simulink model "r23_512p_fft"  (R2026b)
settings: Solver=FixedStepDiscrete  StopTime=5e-5*(127-1)  FixedStep=5e-5
libraries: dspsrcs4 x8
(part 1 of 3)
settings Model: Creator=bzwang_admin  LastModifiedBy=bzwang
settings OptimizationCC: BlockReduction=off  ConditionallyExecuteInputs=off  DefaultParameterBehavior=Inlined  OptimizeBlockIOStorage=off
settings HardwareCC: ProdEndianess=Unspecified  ProdEqTarget=off  ProdHWDeviceType=ASIC/FPGA->ASIC/FPGA  ProdIntDivRoundTo=Undefined  ProdLargestAtomicFloat=None  TargetEndianess=LittleEndian  TargetHWDeviceType=Custom Processor->MATLAB Host Computer  TargetIntDivRoundTo=Zero  TargetLongLongMode=on
settings RTWCC: GenerateReport=on  LaunchReport=on  PackageGeneratedCodeAndArtifacts=on
settings CodeAppCC: ForceParamTrailComments=on  MATLABSourceComments=on  StateflowObjectComments=on

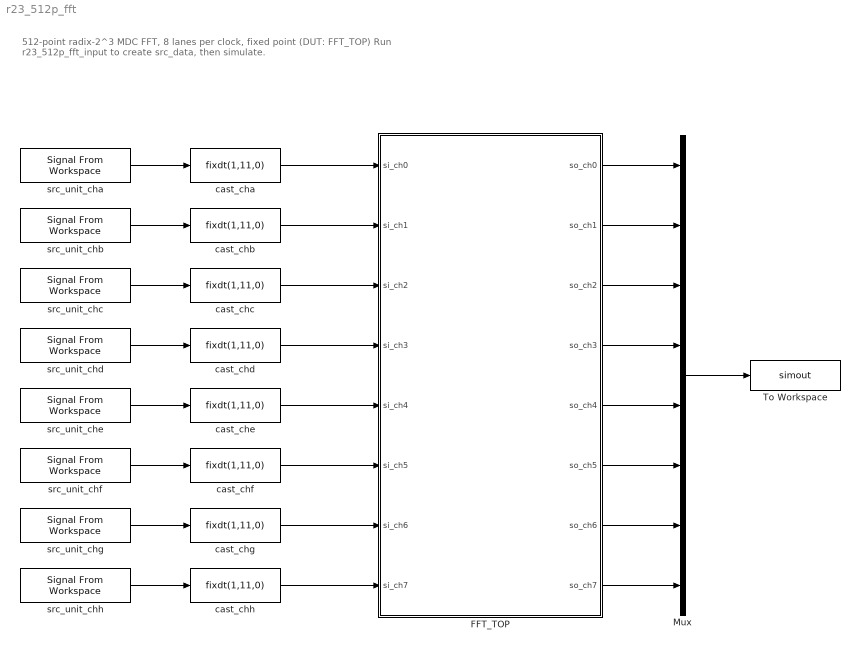
== system r23_512p_fft ==
  note: 512-point radix-2^3 MDC FFT, 8 lanes per clock, fixed point (DUT: FFT_TOP)
      | Run r23_512p_fft_input to create src_data, then simulate.
  FFT_TOP : Subsystem  TreatAsAtomicUnit=on
  Mux : Mux  Inputs=8
  To Workspace : ToWorkspace  VariableName=simout  SampleTime=-1
  cast_cha : DataTypeConversion  OutDataTypeStr=fixdt(1,11,0)  SaturateOnIntegerOverflow=off  RndMeth=Floor
  cast_chb : DataTypeConversion  OutDataTypeStr=fixdt(1,11,0)  SaturateOnIntegerOverflow=off  RndMeth=Floor
  cast_chc : DataTypeConversion  OutDataTypeStr=fixdt(1,11,0)  SaturateOnIntegerOverflow=off  RndMeth=Floor
  cast_chd : DataTypeConversion  OutDataTypeStr=fixdt(1,11,0)  SaturateOnIntegerOverflow=off  RndMeth=Floor
  cast_che : DataTypeConversion  OutDataTypeStr=fixdt(1,11,0)  SaturateOnIntegerOverflow=off  RndMeth=Floor
  cast_chf : DataTypeConversion  OutDataTypeStr=fixdt(1,11,0)  SaturateOnIntegerOverflow=off  RndMeth=Floor
  cast_chg : DataTypeConversion  OutDataTypeStr=fixdt(1,11,0)  SaturateOnIntegerOverflow=off  RndMeth=Floor
  cast_chh : DataTypeConversion  OutDataTypeStr=fixdt(1,11,0)  SaturateOnIntegerOverflow=off  RndMeth=Floor
  src_unit_cha : dspsrcs4/Signal From Workspace  X=src_data.cha  Ts=5e-5  nsamps=1  OutputAfterFinalValue=Setting to zero  ignoreOrWarnInputAndFrameLengths=off  OutputFrames=off
  src_unit_chb : dspsrcs4/Signal From Workspace  X=src_data.chb  Ts=5e-5  nsamps=1  OutputAfterFinalValue=Setting to zero  ignoreOrWarnInputAndFrameLengths=off  OutputFrames=off
  src_unit_chc : dspsrcs4/Signal From Workspace  X=src_data.chc  Ts=5e-5  nsamps=1  OutputAfterFinalValue=Setting to zero  ignoreOrWarnInputAndFrameLengths=off  OutputFrames=off
  src_unit_chd : dspsrcs4/Signal From Workspace  X=src_data.chd  Ts=5e-5  nsamps=1  OutputAfterFinalValue=Setting to zero  ignoreOrWarnInputAndFrameLengths=off  OutputFrames=off
  src_unit_che : dspsrcs4/Signal From Workspace  X=src_data.che  Ts=5e-5  nsamps=1  OutputAfterFinalValue=Setting to zero  ignoreOrWarnInputAndFrameLengths=off  OutputFrames=off
  src_unit_chf : dspsrcs4/Signal From Workspace  X=src_data.chf  Ts=5e-5  nsamps=1  OutputAfterFinalValue=Setting to zero  ignoreOrWarnInputAndFrameLengths=off  OutputFrames=off
  src_unit_chg : dspsrcs4/Signal From Workspace  X=src_data.chg  Ts=5e-5  nsamps=1  OutputAfterFinalValue=Setting to zero  ignoreOrWarnInputAndFrameLengths=off  OutputFrames=off
  src_unit_chh : dspsrcs4/Signal From Workspace  X=src_data.chh  Ts=5e-5  nsamps=1  OutputAfterFinalValue=Setting to zero  ignoreOrWarnInputAndFrameLengths=off  OutputFrames=off
  wires:
  src_unit_cha/1 -> cast_cha/1
  cast_cha/1 -> FFT_TOP/1(si_ch0)
  FFT_TOP/1(so_ch0) -> Mux/1
  src_unit_chb/1 -> cast_chb/1
  cast_chb/1 -> FFT_TOP/2(si_ch1)
  FFT_TOP/2(so_ch1) -> Mux/2
  src_unit_chc/1 -> cast_chc/1
  cast_chc/1 -> FFT_TOP/3(si_ch2)
  FFT_TOP/3(so_ch2) -> Mux/3
  src_unit_chd/1 -> cast_chd/1
  cast_chd/1 -> FFT_TOP/4(si_ch3)
  FFT_TOP/4(so_ch3) -> Mux/4
  src_unit_che/1 -> cast_che/1
  cast_che/1 -> FFT_TOP/5(si_ch4)
  FFT_TOP/5(so_ch4) -> Mux/5
  src_unit_chf/1 -> cast_chf/1
  cast_chf/1 -> FFT_TOP/6(si_ch5)
  FFT_TOP/6(so_ch5) -> Mux/6
  src_unit_chg/1 -> cast_chg/1
  cast_chg/1 -> FFT_TOP/7(si_ch6)
  FFT_TOP/7(so_ch6) -> Mux/7
  src_unit_chh/1 -> cast_chh/1
  cast_chh/1 -> FFT_TOP/8(si_ch7)
  FFT_TOP/8(so_ch7) -> Mux/8
  Mux/1 -> To Workspace/1

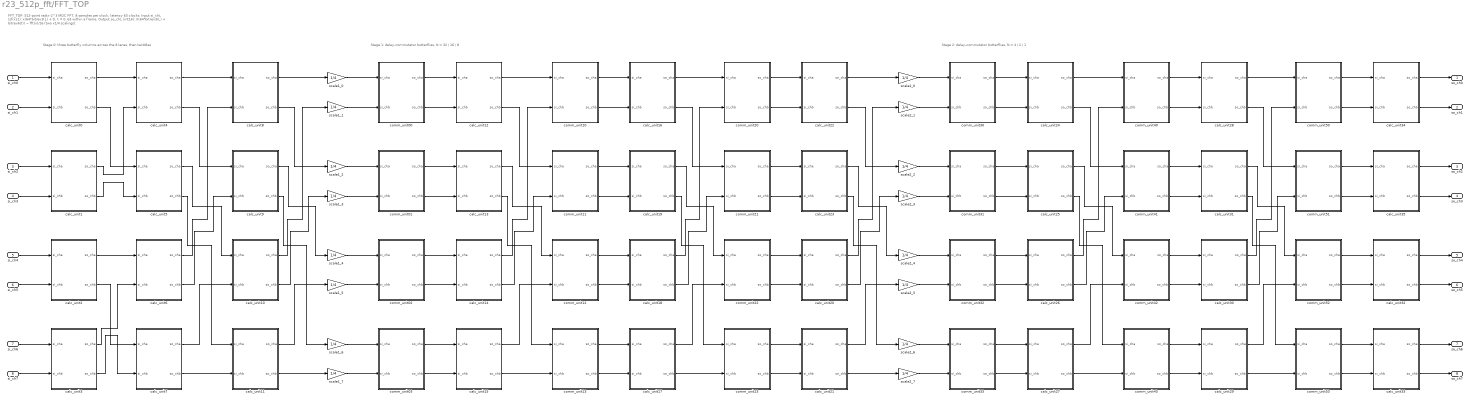
== system r23_512p_fft/FFT_TOP ==
  note: Stage 2: delay-commutator butterflies, N = 4 / 2 / 1
  note: Stage 1: delay-commutator butterflies, N = 32 / 16 / 8
  note: Stage 0: three butterfly columns across the 8 lanes, then twiddles
  note: FFT_TOP: 512-point radix-2^3 MDC FFT, 8 samples per clock, latency 63 clocks.
      | Input  si_chL (sfix11): x(64*bitrev3(L) + t), t = 0..63 within a frame.
      | Output so_chL (int16):  X(64*bitrev3(L) + bitrev6(t)) ~ fft(x)/16 (two x1/4 scalings).
  si_ch0 : Inport
  si_ch1 : Inport  Port=2
  si_ch2 : Inport  Port=3
  si_ch3 : Inport  Port=4
  si_ch4 : Inport  Port=5
  si_ch5 : Inport  Port=6
  si_ch6 : Inport  Port=7
  si_ch7 : Inport  Port=8
  calc_unit0 : Subsystem
  calc_unit1 : Subsystem
  calc_unit10 : Subsystem
  calc_unit11 : Subsystem
  calc_unit12 : Subsystem
  calc_unit13 : Subsystem
  calc_unit14 : Subsystem
  calc_unit15 : Subsystem
  calc_unit16 : Subsystem
  calc_unit17 : Subsystem
  calc_unit18 : Subsystem
  calc_unit19 : Subsystem
  calc_unit2 : Subsystem
  calc_unit20 : Subsystem
  calc_unit21 : Subsystem
  calc_unit22 : Subsystem
  calc_unit23 : Subsystem
  calc_unit24 : Subsystem
  calc_unit25 : Subsystem
  calc_unit26 : Subsystem
  calc_unit27 : Subsystem
  calc_unit28 : Subsystem
  calc_unit29 : Subsystem
  calc_unit3 : Subsystem
  calc_unit30 : Subsystem
  calc_unit31 : Subsystem
  calc_unit32 : Subsystem
  calc_unit33 : Subsystem
  calc_unit34 : Subsystem
  calc_unit35 : Subsystem
  calc_unit4 : Subsystem
  calc_unit5 : Subsystem
  calc_unit6 : Subsystem
  calc_unit7 : Subsystem
  calc_unit8 : Subsystem
  calc_unit9 : Subsystem
  comm_unit00 : Subsystem
      settings: AttributesFormatString=N = 32
  comm_unit01 : Subsystem
      settings: AttributesFormatString=N = 32
  comm_unit02 : Subsystem
      settings: AttributesFormatString=N = 32
  comm_unit03 : Subsystem
      settings: AttributesFormatString=N = 32
  comm_unit10 : Subsystem
      settings: AttributesFormatString=N = 16
  comm_unit11 : Subsystem
      settings: AttributesFormatString=N = 16
  comm_unit12 : Subsystem
      settings: AttributesFormatString=N = 16
  comm_unit13 : Subsystem
      settings: AttributesFormatString=N = 16
  comm_unit20 : Subsystem
      settings: AttributesFormatString=N = 8
  comm_unit21 : Subsystem
      settings: AttributesFormatString=N = 8
  comm_unit22 : Subsystem
      settings: AttributesFormatString=N = 8
  comm_unit23 : Subsystem
      settings: AttributesFormatString=N = 8
  comm_unit30 : Subsystem
      settings: AttributesFormatString=N = 4
  comm_unit31 : Subsystem
      settings: AttributesFormatString=N = 4
  comm_unit32 : Subsystem
      settings: AttributesFormatString=N = 4
  comm_unit33 : Subsystem
      settings: AttributesFormatString=N = 4
  comm_unit40 : Subsystem
      settings: AttributesFormatString=N = 2
  comm_unit41 : Subsystem
      settings: AttributesFormatString=N = 2
  comm_unit42 : Subsystem
      settings: AttributesFormatString=N = 2
  comm_unit43 : Subsystem
      settings: AttributesFormatString=N = 2
  comm_unit50 : Subsystem
      settings: AttributesFormatString=N = 1
  comm_unit51 : Subsystem
      settings: AttributesFormatString=N = 1
  comm_unit52 : Subsystem
      settings: AttributesFormatString=N = 1
  comm_unit53 : Subsystem
      settings: AttributesFormatString=N = 1
  scale1_{0..7} (8 alike) : Gain  Gain=1/4  OutDataTypeStr=fixdt(1,12,0)  RndMeth=Nearest
  scale2_{0..7} (8 alike) : Gain  Gain=1/4  OutDataTypeStr=fixdt(1,13,0)  RndMeth=Nearest
  so_ch0 : Outport
  so_ch1 : Outport  Port=2
  so_ch2 : Outport  Port=3
  so_ch3 : Outport  Port=4
  so_ch4 : Outport  Port=5
  so_ch5 : Outport  Port=6
  so_ch6 : Outport  Port=7
  so_ch7 : Outport  Port=8
  wires:
  calc_unit34/2(so_chb) -> so_ch1/1
  calc_unit21/2(so_chb) -> scale2_7/1
  scale1_7/1 -> comm_unit03/2(si_chb)
  scale1_1/1 -> comm_unit00/2(si_chb)
  calc_unit35/2(so_chb) -> so_ch3/1
  calc_unit8/1(so_cha) -> scale1_0/1
  calc_unit32/1(so_cha) -> so_ch4/1
  scale1_2/1 -> comm_unit01/1(si_cha)
  calc_unit30/2(so_chb) -> comm_unit51/2(si_chb)
  calc_unit9/1(so_cha) -> scale1_4/1
  scale1_0/1 -> comm_unit00/1(si_cha)
  comm_unit13/2(so_chb) -> calc_unit17/2(si_chb)
  calc_unit33/2(so_chb) -> so_ch7/1
  calc_unit33/1(so_cha) -> so_ch6/1
  calc_unit8/2(so_chb) -> scale1_2/1
  scale1_3/1 -> comm_unit01/2(si_chb)
  comm_unit23/1(so_cha) -> calc_unit21/1(si_cha)
  calc_unit2/1(so_cha) -> calc_unit6/1(si_cha)
  comm_unit22/1(so_cha) -> calc_unit20/1(si_cha)
  scale1_4/1 -> comm_unit02/1(si_cha)
  calc_unit29/1(so_cha) -> comm_unit52/2(si_chb)
  scale1_5/1 -> comm_unit02/2(si_chb)
  comm_unit10/2(so_chb) -> calc_unit16/2(si_chb)
  si_ch7/1 -> calc_unit3/2(si_chb)
  scale1_6/1 -> comm_unit03/1(si_cha)
  calc_unit11/1(so_cha) -> scale1_5/1
  calc_unit10/1(so_cha) -> scale1_1/1
  si_ch5/1 -> calc_unit2/2(si_chb)
  scale2_2/1 -> comm_unit31/1(si_cha)
  comm_unit43/2(so_chb) -> calc_unit29/2(si_chb)
  calc_unit7/2(so_chb) -> calc_unit11/2(si_chb)
  calc_unit30/1(so_cha) -> comm_unit50/2(si_chb)
  comm_unit02/1(so_cha) -> calc_unit14/1(si_cha)
  si_ch4/1 -> calc_unit2/1(si_cha)
  comm_unit12/1(so_cha) -> calc_unit18/1(si_cha)
  calc_unit11/2(so_chb) -> scale1_7/1
  calc_unit10/2(so_chb) -> scale1_3/1
  calc_unit9/2(so_chb) -> scale1_6/1
  scale2_3/1 -> comm_unit31/2(si_chb)
  scale2_5/1 -> comm_unit32/2(si_chb)
  calc_unit15/1(so_cha) -> comm_unit12/2(si_chb)
  si_ch6/1 -> calc_unit3/1(si_cha)
  scale2_7/1 -> comm_unit33/2(si_chb)
  scale2_4/1 -> comm_unit32/1(si_cha)
  scale2_6/1 -> comm_unit33/1(si_cha)
  comm_unit22/2(so_chb) -> calc_unit20/2(si_chb)
  calc_unit22/2(so_chb) -> scale2_2/1
  comm_unit01/1(so_cha) -> calc_unit13/1(si_cha)
  comm_unit12/2(so_chb) -> calc_unit18/2(si_chb)
  calc_unit20/1(so_cha) -> scale2_1/1
  comm_unit21/1(so_cha) -> calc_unit23/1(si_cha)
  calc_unit22/1(so_cha) -> scale2_0/1
  calc_unit28/1(so_cha) -> comm_unit50/1(si_cha)
  si_ch2/1 -> calc_unit1/1(si_cha)
  comm_unit42/1(so_cha) -> calc_unit30/1(si_cha)
  scale2_0/1 -> comm_unit30/1(si_cha)
  comm_unit02/2(so_chb) -> calc_unit14/2(si_chb)
  comm_unit21/2(so_chb) -> calc_unit23/2(si_chb)
  comm_unit11/1(so_cha) -> calc_unit19/1(si_cha)
  comm_unit13/1(so_cha) -> calc_unit17/1(si_cha)
  comm_unit10/1(so_cha) -> calc_unit16/1(si_cha)
  comm_unit01/2(so_chb) -> calc_unit13/2(si_chb)
  comm_unit23/2(so_chb) -> calc_unit21/2(si_chb)
  calc_unit23/2(so_chb) -> scale2_6/1
  calc_unit31/2(so_chb) -> comm_unit53/1(si_cha)
  comm_unit32/2(so_chb) -> calc_unit26/2(si_chb)
  calc_unit23/1(so_cha) -> scale2_4/1
  calc_unit21/1(so_cha) -> scale2_5/1
  calc_unit27/2(so_chb) -> comm_unit43/2(si_chb)
  calc_unit20/2(so_chb) -> scale2_3/1
  calc_unit24/1(so_cha) -> comm_unit40/1(si_cha)
  si_ch3/1 -> calc_unit1/2(si_chb)
  calc_unit7/1(so_cha) -> calc_unit10/2(si_chb)
  comm_unit50/1(so_cha) -> calc_unit34/1(si_cha)
  calc_unit27/1(so_cha) -> comm_unit42/2(si_chb)
  calc_unit35/1(so_cha) -> so_ch2/1
  si_ch1/1 -> calc_unit0/2(si_chb)
  comm_unit52/2(so_chb) -> calc_unit32/2(si_chb)
  si_ch0/1 -> calc_unit0/1(si_cha)
  comm_unit30/1(so_cha) -> calc_unit24/1(si_cha)
  comm_unit20/2(so_chb) -> calc_unit22/2(si_chb)
  comm_unit50/2(so_chb) -> calc_unit34/2(si_chb)
  calc_unit12/1(so_cha) -> comm_unit10/1(si_cha)
  comm_unit42/2(so_chb) -> calc_unit30/2(si_chb)
  calc_unit3/1(so_cha) -> calc_unit6/2(si_chb)
  comm_unit33/2(so_chb) -> calc_unit27/2(si_chb)
  comm_unit03/1(so_cha) -> calc_unit15/1(si_cha)
  comm_unit41/1(so_cha) -> calc_unit31/1(si_cha)
  comm_unit20/1(so_cha) -> calc_unit22/1(si_cha)
  comm_unit00/1(so_cha) -> calc_unit12/1(si_cha)
  comm_unit53/2(so_chb) -> calc_unit33/2(si_chb)
  calc_unit1/2(so_chb) -> calc_unit5/2(si_chb)
  comm_unit40/2(so_chb) -> calc_unit28/2(si_chb)
  comm_unit32/1(so_cha) -> calc_unit26/1(si_cha)
  calc_unit6/2(so_chb) -> calc_unit9/2(si_chb)
  comm_unit43/1(so_cha) -> calc_unit29/1(si_cha)
  calc_unit16/1(so_cha) -> comm_unit20/1(si_cha)
  calc_unit16/2(so_chb) -> comm_unit21/1(si_cha)
  calc_unit34/1(so_cha) -> so_ch0/1
  calc_unit17/2(so_chb) -> comm_unit23/2(si_chb)
  calc_unit4/2(so_chb) -> calc_unit9/1(si_cha)
  calc_unit32/2(so_chb) -> so_ch5/1
  calc_unit13/2(so_chb) -> comm_unit13/1(si_cha)
  calc_unit3/2(so_chb) -> calc_unit7/2(si_chb)
  calc_unit14/2(so_chb) -> comm_unit11/2(si_chb)
  calc_unit12/2(so_chb) -> comm_unit11/1(si_cha)
  calc_unit14/1(so_cha) -> comm_unit10/2(si_chb)
  calc_unit1/1(so_cha) -> calc_unit4/2(si_chb)
  calc_unit13/1(so_cha) -> comm_unit12/1(si_cha)
  comm_unit11/2(so_chb) -> calc_unit19/2(si_chb)
  calc_unit18/1(so_cha) -> comm_unit20/2(si_chb)
  comm_unit03/2(so_chb) -> calc_unit15/2(si_chb)
  comm_unit40/1(so_cha) -> calc_unit28/1(si_cha)
  calc_unit28/2(so_chb) -> comm_unit51/1(si_cha)
  comm_unit52/1(so_cha) -> calc_unit32/1(si_cha)
  calc_unit2/2(so_chb) -> calc_unit7/1(si_cha)
  calc_unit0/1(so_cha) -> calc_unit4/1(si_cha)
  calc_unit19/1(so_cha) -> comm_unit22/1(si_cha)
  comm_unit53/1(so_cha) -> calc_unit33/1(si_cha)
  calc_unit26/2(so_chb) -> comm_unit41/2(si_chb)
  calc_unit18/2(so_chb) -> comm_unit21/2(si_chb)
  comm_unit31/1(so_cha) -> calc_unit25/1(si_cha)
  calc_unit25/2(so_chb) -> comm_unit43/1(si_cha)
  comm_unit00/2(so_chb) -> calc_unit12/2(si_chb)
  calc_unit26/1(so_cha) -> comm_unit40/2(si_chb)
  calc_unit5/2(so_chb) -> calc_unit11/1(si_cha)
  calc_unit19/2(so_chb) -> comm_unit23/1(si_cha)
  calc_unit25/1(so_cha) -> comm_unit42/1(si_cha)
  comm_unit30/2(so_chb) -> calc_unit24/2(si_chb)
  calc_unit24/2(so_chb) -> comm_unit41/1(si_cha)
  comm_unit33/1(so_cha) -> calc_unit27/1(si_cha)
  calc_unit17/1(so_cha) -> comm_unit22/2(si_chb)
  scale2_1/1 -> comm_unit30/2(si_chb)
  calc_unit5/1(so_cha) -> calc_unit10/1(si_cha)
  calc_unit29/2(so_chb) -> comm_unit53/2(si_chb)
  calc_unit15/2(so_chb) -> comm_unit13/2(si_chb)
  comm_unit41/2(so_chb) -> calc_unit31/2(si_chb)
  comm_unit51/2(so_chb) -> calc_unit35/2(si_chb)
  calc_unit31/1(so_cha) -> comm_unit52/1(si_cha)
  comm_unit51/1(so_cha) -> calc_unit35/1(si_cha)
  calc_unit6/1(so_cha) -> calc_unit8/2(si_chb)
  calc_unit4/1(so_cha) -> calc_unit8/1(si_cha)
  comm_unit31/2(so_chb) -> calc_unit25/2(si_chb)
  calc_unit0/2(so_chb) -> calc_unit5/1(si_cha)

== system r23_512p_fft/FFT_TOP/calc_unit0 ==
  si_cha : Inport
  si_chb : Inport  Port=2
  r2_unit : MATLAB Function  TreatAsAtomicUnit=on
  so_cha : Outport
  so_chb : Outport  Port=2
  wires:
  r2_unit/2(so_chb) -> so_chb/1
  si_chb/1 -> r2_unit/2(si_chb)
  si_cha/1 -> r2_unit/1(si_cha)
  r2_unit/1(so_cha) -> so_cha/1

== system r23_512p_fft/FFT_TOP/calc_unit1 ==
  si_cha : Inport
  si_chb : Inport  Port=2
  bwr_unit : MATLAB Function  TreatAsAtomicUnit=on
      settings: AttributesFormatString=W^0 | W^128
  r2_unit : MATLAB Function  TreatAsAtomicUnit=on
  so_cha : Outport
  so_chb : Outport  Port=2
  wires:
  bwr_unit/1(so_cha) -> so_cha/1
  r2_unit/2(so_chb) -> bwr_unit/2(si_chb)
  si_cha/1 -> r2_unit/1(si_cha)
  r2_unit/1(so_cha) -> bwr_unit/1(si_cha)
  si_chb/1 -> r2_unit/2(si_chb)
  bwr_unit/2(so_chb) -> so_chb/1

== system r23_512p_fft/FFT_TOP/calc_unit10 ==
  si_cha : Inport
  si_chb : Inport  Port=2
  bwr_unit : MATLAB Function  TreatAsAtomicUnit=on
      settings: AttributesFormatString=W^(1k) | W^(5k)
  r2_unit : MATLAB Function  TreatAsAtomicUnit=on
  so_cha : Outport
  so_chb : Outport  Port=2
  wires:
  bwr_unit/2(so_chb) -> so_chb/1
  si_chb/1 -> r2_unit/2(si_chb)
  r2_unit/1(so_cha) -> bwr_unit/1(si_cha)
  si_cha/1 -> r2_unit/1(si_cha)
  r2_unit/2(so_chb) -> bwr_unit/2(si_chb)
  bwr_unit/1(so_cha) -> so_cha/1

== system r23_512p_fft/FFT_TOP/calc_unit11 ==
  si_cha : Inport
  si_chb : Inport  Port=2
  bwr_unit : MATLAB Function  TreatAsAtomicUnit=on
      settings: AttributesFormatString=W^(3k) | W^(7k)
  r2_unit : MATLAB Function  TreatAsAtomicUnit=on
  so_cha : Outport
  so_chb : Outport  Port=2
  wires:
  bwr_unit/1(so_cha) -> so_cha/1
  r2_unit/2(so_chb) -> bwr_unit/2(si_chb)
  si_cha/1 -> r2_unit/1(si_cha)
  r2_unit/1(so_cha) -> bwr_unit/1(si_cha)
  si_chb/1 -> r2_unit/2(si_chb)
  bwr_unit/2(so_chb) -> so_chb/1

== system r23_512p_fft/FFT_TOP/calc_unit12 ==
  si_cha : Inport
  si_chb : Inport  Port=2
  r2_unit : MATLAB Function  TreatAsAtomicUnit=on
  so_cha : Outport
  so_chb : Outport  Port=2
  wires:
  r2_unit/2(so_chb) -> so_chb/1
  si_chb/1 -> r2_unit/2(si_chb)
  si_cha/1 -> r2_unit/1(si_cha)
  r2_unit/1(so_cha) -> so_cha/1

== system r23_512p_fft/FFT_TOP/calc_unit13 ==
  si_cha : Inport
  si_chb : Inport  Port=2
  r2_unit : MATLAB Function  TreatAsAtomicUnit=on
  so_cha : Outport
  so_chb : Outport  Port=2
  wires:
  r2_unit/1(so_cha) -> so_cha/1
  si_cha/1 -> r2_unit/1(si_cha)
  si_chb/1 -> r2_unit/2(si_chb)
  r2_unit/2(so_chb) -> so_chb/1

== system r23_512p_fft/FFT_TOP/calc_unit14 ==
  si_cha : Inport
  si_chb : Inport  Port=2
  r2_unit : MATLAB Function  TreatAsAtomicUnit=on
  so_cha : Outport
  so_chb : Outport  Port=2
  wires:
  r2_unit/2(so_chb) -> so_chb/1
  si_chb/1 -> r2_unit/2(si_chb)
  si_cha/1 -> r2_unit/1(si_cha)
  r2_unit/1(so_cha) -> so_cha/1

== system r23_512p_fft/FFT_TOP/calc_unit15 ==
  si_cha : Inport
  si_chb : Inport  Port=2
  r2_unit : MATLAB Function  TreatAsAtomicUnit=on
  so_cha : Outport
  so_chb : Outport  Port=2
  wires:
  r2_unit/1(so_cha) -> so_cha/1
  si_cha/1 -> r2_unit/1(si_cha)
  si_chb/1 -> r2_unit/2(si_chb)
  r2_unit/2(so_chb) -> so_chb/1

== system r23_512p_fft/FFT_TOP/calc_unit16 ==
  si_cha : Inport
  si_chb : Inport  Port=2
  r2_unit : MATLAB Function  TreatAsAtomicUnit=on
  so_cha : Outport
  so_chb : Outport  Port=2
  wires:
  r2_unit/2(so_chb) -> so_chb/1
  si_chb/1 -> r2_unit/2(si_chb)
  si_cha/1 -> r2_unit/1(si_cha)
  r2_unit/1(so_cha) -> so_cha/1

== system r23_512p_fft/FFT_TOP/calc_unit17 ==
  si_cha : Inport
  si_chb : Inport  Port=2
  pwr_unit : MATLAB Function  TreatAsAtomicUnit=on
      settings: AttributesFormatString=W^0 | W^128
  r2_unit : MATLAB Function  TreatAsAtomicUnit=on
  so_cha : Outport
  so_chb : Outport  Port=2
  wires:
  r2_unit/1(so_cha) -> so_cha/1
  pwr_unit/1(so_cha) -> r2_unit/1(si_cha)
  si_cha/1 -> pwr_unit/1(si_cha)
  pwr_unit/2(so_chb) -> r2_unit/2(si_chb)
  r2_unit/2(so_chb) -> so_chb/1
  si_chb/1 -> pwr_unit/2(si_chb)

== system r23_512p_fft/FFT_TOP/calc_unit18 ==
  si_cha : Inport
  si_chb : Inport  Port=2
  r2_unit : MATLAB Function  TreatAsAtomicUnit=on
  so_cha : Outport
  so_chb : Outport  Port=2
  wires:
  r2_unit/1(so_cha) -> so_cha/1
  si_cha/1 -> r2_unit/1(si_cha)
  si_chb/1 -> r2_unit/2(si_chb)
  r2_unit/2(so_chb) -> so_chb/1

== system r23_512p_fft/FFT_TOP/calc_unit19 ==
  si_cha : Inport
  si_chb : Inport  Port=2
  pwr_unit : MATLAB Function  TreatAsAtomicUnit=on
      settings: AttributesFormatString=W^0 | W^128
  r2_unit : MATLAB Function  TreatAsAtomicUnit=on
  so_cha : Outport
  so_chb : Outport  Port=2
  wires:
  r2_unit/1(so_cha) -> so_cha/1
  pwr_unit/1(so_cha) -> r2_unit/1(si_cha)
  si_cha/1 -> pwr_unit/1(si_cha)
  pwr_unit/2(so_chb) -> r2_unit/2(si_chb)
  r2_unit/2(so_chb) -> so_chb/1
  si_chb/1 -> pwr_unit/2(si_chb)

== system r23_512p_fft/FFT_TOP/calc_unit2 ==
  si_cha : Inport
  si_chb : Inport  Port=2
  r2_unit : MATLAB Function  TreatAsAtomicUnit=on
  so_cha : Outport
  so_chb : Outport  Port=2
  wires:
  r2_unit/2(so_chb) -> so_chb/1
  si_chb/1 -> r2_unit/2(si_chb)
  si_cha/1 -> r2_unit/1(si_cha)
  r2_unit/1(so_cha) -> so_cha/1

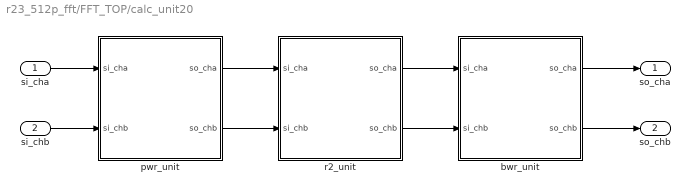
== system r23_512p_fft/FFT_TOP/calc_unit20 ==
  si_cha : Inport
  si_chb : Inport  Port=2
  bwr_unit : MATLAB Function  TreatAsAtomicUnit=on
      settings: AttributesFormatString=W^(8k) | W^(40k)
  pwr_unit : MATLAB Function  TreatAsAtomicUnit=on
      settings: AttributesFormatString=W^0 | W^64
  r2_unit : MATLAB Function  TreatAsAtomicUnit=on
  so_cha : Outport
  so_chb : Outport  Port=2
  wires:
  bwr_unit/1(so_cha) -> so_cha/1
  r2_unit/2(so_chb) -> bwr_unit/2(si_chb)
  pwr_unit/1(so_cha) -> r2_unit/1(si_cha)
  r2_unit/1(so_cha) -> bwr_unit/1(si_cha)
  si_cha/1 -> pwr_unit/1(si_cha)
  pwr_unit/2(so_chb) -> r2_unit/2(si_chb)
  bwr_unit/2(so_chb) -> so_chb/1
  si_chb/1 -> pwr_unit/2(si_chb)

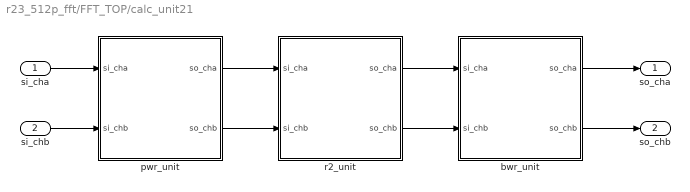
== system r23_512p_fft/FFT_TOP/calc_unit21 ==
  si_cha : Inport
  si_chb : Inport  Port=2
  bwr_unit : MATLAB Function  TreatAsAtomicUnit=on
      settings: AttributesFormatString=W^(24k) | W^(56k)
  pwr_unit : MATLAB Function  TreatAsAtomicUnit=on
      settings: AttributesFormatString=W^0 | W^192
  r2_unit : MATLAB Function  TreatAsAtomicUnit=on
  so_cha : Outport
  so_chb : Outport  Port=2
  wires:
  si_chb/1 -> pwr_unit/2(si_chb)
  bwr_unit/2(so_chb) -> so_chb/1
  pwr_unit/2(so_chb) -> r2_unit/2(si_chb)
  si_cha/1 -> pwr_unit/1(si_cha)
  r2_unit/1(so_cha) -> bwr_unit/1(si_cha)
  pwr_unit/1(so_cha) -> r2_unit/1(si_cha)
  r2_unit/2(so_chb) -> bwr_unit/2(si_chb)
  bwr_unit/1(so_cha) -> so_cha/1

== system r23_512p_fft/FFT_TOP/calc_unit22 ==
  si_cha : Inport
  si_chb : Inport  Port=2
  bwr_unit : MATLAB Function  TreatAsAtomicUnit=on
      settings: AttributesFormatString=W^0 | W^(32k)
  r2_unit : MATLAB Function  TreatAsAtomicUnit=on
  so_cha : Outport
  so_chb : Outport  Port=2
  wires:
  bwr_unit/1(so_cha) -> so_cha/1
  r2_unit/2(so_chb) -> bwr_unit/2(si_chb)
  si_cha/1 -> r2_unit/1(si_cha)
  r2_unit/1(so_cha) -> bwr_unit/1(si_cha)
  si_chb/1 -> r2_unit/2(si_chb)
  bwr_unit/2(so_chb) -> so_chb/1

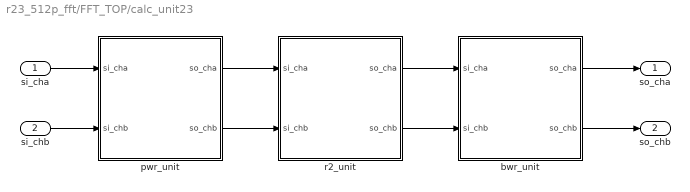
== system r23_512p_fft/FFT_TOP/calc_unit23 ==
  si_cha : Inport
  si_chb : Inport  Port=2
  bwr_unit : MATLAB Function  TreatAsAtomicUnit=on
      settings: AttributesFormatString=W^(16k) | W^(48k)
  pwr_unit : MATLAB Function  TreatAsAtomicUnit=on
      settings: AttributesFormatString=W^0 | W^128
  r2_unit : MATLAB Function  TreatAsAtomicUnit=on
  so_cha : Outport
  so_chb : Outport  Port=2
  wires:
  si_chb/1 -> pwr_unit/2(si_chb)
  bwr_unit/2(so_chb) -> so_chb/1
  pwr_unit/2(so_chb) -> r2_unit/2(si_chb)
  si_cha/1 -> pwr_unit/1(si_cha)
  r2_unit/1(so_cha) -> bwr_unit/1(si_cha)
  pwr_unit/1(so_cha) -> r2_unit/1(si_cha)
  r2_unit/2(so_chb) -> bwr_unit/2(si_chb)
  bwr_unit/1(so_cha) -> so_cha/1

== system r23_512p_fft/FFT_TOP/calc_unit24 ==
  si_cha : Inport
  si_chb : Inport  Port=2
  r2_unit : MATLAB Function  TreatAsAtomicUnit=on
  so_cha : Outport
  so_chb : Outport  Port=2
  wires:
  r2_unit/1(so_cha) -> so_cha/1
  si_cha/1 -> r2_unit/1(si_cha)
  si_chb/1 -> r2_unit/2(si_chb)
  r2_unit/2(so_chb) -> so_chb/1

== system r23_512p_fft/FFT_TOP/calc_unit25 ==
  si_cha : Inport
  si_chb : Inport  Port=2
  r2_unit : MATLAB Function  TreatAsAtomicUnit=on
  so_cha : Outport
  so_chb : Outport  Port=2
  wires:
  si_chb/1 -> r2_unit/2(si_chb)
  r2_unit/2(so_chb) -> so_chb/1
  si_cha/1 -> r2_unit/1(si_cha)
  r2_unit/1(so_cha) -> so_cha/1

== system r23_512p_fft/FFT_TOP/calc_unit26 ==
  si_cha : Inport
  si_chb : Inport  Port=2
  r2_unit : MATLAB Function  TreatAsAtomicUnit=on
  so_cha : Outport
  so_chb : Outport  Port=2
  wires:
  r2_unit/1(so_cha) -> so_cha/1
  si_cha/1 -> r2_unit/1(si_cha)
  r2_unit/2(so_chb) -> so_chb/1
  si_chb/1 -> r2_unit/2(si_chb)

== system r23_512p_fft/FFT_TOP/calc_unit27 ==
  si_cha : Inport
  si_chb : Inport  Port=2
  r2_unit : MATLAB Function  TreatAsAtomicUnit=on
  so_cha : Outport
  so_chb : Outport  Port=2
  wires:
  si_chb/1 -> r2_unit/2(si_chb)
  r2_unit/2(so_chb) -> so_chb/1
  si_cha/1 -> r2_unit/1(si_cha)
  r2_unit/1(so_cha) -> so_cha/1

== system r23_512p_fft/FFT_TOP/calc_unit28 ==
  si_cha : Inport
  si_chb : Inport  Port=2
  r2_unit : MATLAB Function  TreatAsAtomicUnit=on
  so_cha : Outport
  so_chb : Outport  Port=2
  wires:
  r2_unit/1(so_cha) -> so_cha/1
  si_cha/1 -> r2_unit/1(si_cha)
  si_chb/1 -> r2_unit/2(si_chb)
  r2_unit/2(so_chb) -> so_chb/1

== system r23_512p_fft/FFT_TOP/calc_unit29 ==
  si_cha : Inport
  si_chb : Inport  Port=2
  pwr_unit : MATLAB Function  TreatAsAtomicUnit=on
      settings: AttributesFormatString=W^0 | W^128
  r2_unit : MATLAB Function  TreatAsAtomicUnit=on
  so_cha : Outport
  so_chb : Outport  Port=2
  wires:
  si_chb/1 -> pwr_unit/2(si_chb)
  r2_unit/2(so_chb) -> so_chb/1
  pwr_unit/2(so_chb) -> r2_unit/2(si_chb)
  si_cha/1 -> pwr_unit/1(si_cha)
  pwr_unit/1(so_cha) -> r2_unit/1(si_cha)
  r2_unit/1(so_cha) -> so_cha/1

== system r23_512p_fft/FFT_TOP/calc_unit3 ==
  si_cha : Inport
  si_chb : Inport  Port=2
  bwr_unit : MATLAB Function  TreatAsAtomicUnit=on
      settings: AttributesFormatString=W^0 | W^128
  r2_unit : MATLAB Function  TreatAsAtomicUnit=on
  so_cha : Outport
  so_chb : Outport  Port=2
  wires:
  r2_unit/2(so_chb) -> bwr_unit/2(si_chb)
  r2_unit/1(so_cha) -> bwr_unit/1(si_cha)
  bwr_unit/1(so_cha) -> so_cha/1
  si_cha/1 -> r2_unit/1(si_cha)
  si_chb/1 -> r2_unit/2(si_chb)
  bwr_unit/2(so_chb) -> so_chb/1

== system r23_512p_fft/FFT_TOP/calc_unit30 ==
  si_cha : Inport
  si_chb : Inport  Port=2
  r2_unit : MATLAB Function  TreatAsAtomicUnit=on
  so_cha : Outport
  so_chb : Outport  Port=2
  wires:
  si_chb/1 -> r2_unit/2(si_chb)
  r2_unit/2(so_chb) -> so_chb/1
  si_cha/1 -> r2_unit/1(si_cha)
  r2_unit/1(so_cha) -> so_cha/1

== system r23_512p_fft/FFT_TOP/calc_unit31 ==
  si_cha : Inport
  si_chb : Inport  Port=2
  pwr_unit : MATLAB Function  TreatAsAtomicUnit=on
      settings: AttributesFormatString=W^0 | W^128
  r2_unit : MATLAB Function  TreatAsAtomicUnit=on
  so_cha : Outport
  so_chb : Outport  Port=2
  wires:
  si_chb/1 -> pwr_unit/2(si_chb)
  r2_unit/2(so_chb) -> so_chb/1
  pwr_unit/2(so_chb) -> r2_unit/2(si_chb)
  si_cha/1 -> pwr_unit/1(si_cha)
  pwr_unit/1(so_cha) -> r2_unit/1(si_cha)
  r2_unit/1(so_cha) -> so_cha/1

== system r23_512p_fft/FFT_TOP/calc_unit32 ==
  si_cha : Inport
  si_chb : Inport  Port=2
  pwr_unit : MATLAB Function  TreatAsAtomicUnit=on
      settings: AttributesFormatString=W^0 | W^64
  r2_unit : MATLAB Function  TreatAsAtomicUnit=on
  so_cha : Outport
  so_chb : Outport  Port=2
  wires:
  r2_unit/2(so_chb) -> so_chb/1
  si_chb/1 -> pwr_unit/2(si_chb)
  pwr_unit/2(so_chb) -> r2_unit/2(si_chb)
  si_cha/1 -> pwr_unit/1(si_cha)
  pwr_unit/1(so_cha) -> r2_unit/1(si_cha)
  r2_unit/1(so_cha) -> so_cha/1

== system r23_512p_fft/FFT_TOP/calc_unit33 ==
  si_cha : Inport
  si_chb : Inport  Port=2
  pwr_unit : MATLAB Function  TreatAsAtomicUnit=on
      settings: AttributesFormatString=W^0 | W^192
  r2_unit : MATLAB Function  TreatAsAtomicUnit=on
  so_cha : Outport
  so_chb : Outport  Port=2
  wires:
  r2_unit/2(so_chb) -> so_chb/1
  r2_unit/1(so_cha) -> so_cha/1
  pwr_unit/1(so_cha) -> r2_unit/1(si_cha)
  si_cha/1 -> pwr_unit/1(si_cha)
  pwr_unit/2(so_chb) -> r2_unit/2(si_chb)
  si_chb/1 -> pwr_unit/2(si_chb)

== system r23_512p_fft/FFT_TOP/calc_unit34 ==
  si_cha : Inport
  si_chb : Inport  Port=2
  r2_unit : MATLAB Function  TreatAsAtomicUnit=on
  so_cha : Outport
  so_chb : Outport  Port=2
  wires:
  si_chb/1 -> r2_unit/2(si_chb)
  r2_unit/2(so_chb) -> so_chb/1
  si_cha/1 -> r2_unit/1(si_cha)
  r2_unit/1(so_cha) -> so_cha/1

== system r23_512p_fft/FFT_TOP/calc_unit35 ==
  si_cha : Inport
  si_chb : Inport  Port=2
  pwr_unit : MATLAB Function  TreatAsAtomicUnit=on
      settings: AttributesFormatString=W^0 | W^128
  r2_unit : MATLAB Function  TreatAsAtomicUnit=on
  so_cha : Outport
  so_chb : Outport  Port=2
  wires:
  r2_unit/1(so_cha) -> so_cha/1
  pwr_unit/1(so_cha) -> r2_unit/1(si_cha)
  si_cha/1 -> pwr_unit/1(si_cha)
  pwr_unit/2(so_chb) -> r2_unit/2(si_chb)
  r2_unit/2(so_chb) -> so_chb/1
  si_chb/1 -> pwr_unit/2(si_chb)

== system r23_512p_fft/FFT_TOP/calc_unit4 ==
  si_cha : Inport
  si_chb : Inport  Port=2
  r2_unit : MATLAB Function  TreatAsAtomicUnit=on
  so_cha : Outport
  so_chb : Outport  Port=2
  wires:
  r2_unit/1(so_cha) -> so_cha/1
  si_cha/1 -> r2_unit/1(si_cha)
  si_chb/1 -> r2_unit/2(si_chb)
  r2_unit/2(so_chb) -> so_chb/1

== system r23_512p_fft/FFT_TOP/calc_unit5 ==
  si_cha : Inport
  si_chb : Inport  Port=2
  r2_unit : MATLAB Function  TreatAsAtomicUnit=on
  so_cha : Outport
  so_chb : Outport  Port=2
  wires:
  r2_unit/2(so_chb) -> so_chb/1
  si_chb/1 -> r2_unit/2(si_chb)
  si_cha/1 -> r2_unit/1(si_cha)
  r2_unit/1(so_cha) -> so_cha/1

== system r23_512p_fft/FFT_TOP/calc_unit6 ==
  si_cha : Inport
  si_chb : Inport  Port=2
  bwr_unit : MATLAB Function  TreatAsAtomicUnit=on
      settings: AttributesFormatString=W^0 | W^128
  r2_unit : MATLAB Function  TreatAsAtomicUnit=on
  so_cha : Outport
  so_chb : Outport  Port=2
  wires:
  bwr_unit/1(so_cha) -> so_cha/1
  r2_unit/2(so_chb) -> bwr_unit/2(si_chb)
  si_cha/1 -> r2_unit/1(si_cha)
  r2_unit/1(so_cha) -> bwr_unit/1(si_cha)
  si_chb/1 -> r2_unit/2(si_chb)
  bwr_unit/2(so_chb) -> so_chb/1

== system r23_512p_fft/FFT_TOP/calc_unit7 ==
  si_cha : Inport
  si_chb : Inport  Port=2
  bwr_unit : MATLAB Function  TreatAsAtomicUnit=on
      settings: AttributesFormatString=W^64 | W^192
  r2_unit : MATLAB Function  TreatAsAtomicUnit=on
  so_cha : Outport
  so_chb : Outport  Port=2
  wires:
  bwr_unit/2(so_chb) -> so_chb/1
  si_chb/1 -> r2_unit/2(si_chb)
  r2_unit/1(so_cha) -> bwr_unit/1(si_cha)
  si_cha/1 -> r2_unit/1(si_cha)
  r2_unit/2(so_chb) -> bwr_unit/2(si_chb)
  bwr_unit/1(so_cha) -> so_cha/1

== system r23_512p_fft/FFT_TOP/calc_unit8 ==
  si_cha : Inport
  si_chb : Inport  Port=2
  bwr_unit : MATLAB Function  TreatAsAtomicUnit=on
      settings: AttributesFormatString=W^0 | W^(4k)
  r2_unit : MATLAB Function  TreatAsAtomicUnit=on
  so_cha : Outport
  so_chb : Outport  Port=2
  wires:
  bwr_unit/2(so_chb) -> so_chb/1
  si_chb/1 -> r2_unit/2(si_chb)
  r2_unit/1(so_cha) -> bwr_unit/1(si_cha)
  si_cha/1 -> r2_unit/1(si_cha)
  r2_unit/2(so_chb) -> bwr_unit/2(si_chb)
  bwr_unit/1(so_cha) -> so_cha/1

== system r23_512p_fft/FFT_TOP/calc_unit9 ==
  si_cha : Inport
  si_chb : Inport  Port=2
  bwr_unit : MATLAB Function  TreatAsAtomicUnit=on
      settings: AttributesFormatString=W^(2k) | W^(6k)
  r2_unit : MATLAB Function  TreatAsAtomicUnit=on
  so_cha : Outport
  so_chb : Outport  Port=2
  wires:
  bwr_unit/1(so_cha) -> so_cha/1
  r2_unit/2(so_chb) -> bwr_unit/2(si_chb)
  si_cha/1 -> r2_unit/1(si_cha)
  r2_unit/1(so_cha) -> bwr_unit/1(si_cha)
  si_chb/1 -> r2_unit/2(si_chb)
  bwr_unit/2(so_chb) -> so_chb/1

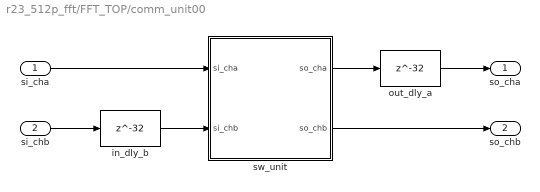
== system r23_512p_fft/FFT_TOP/comm_unit00 ==
  si_cha : Inport
  si_chb : Inport  Port=2
  in_dly_b : Delay  DelayLength=32
  out_dly_a : Delay  DelayLength=32
  sw_unit : MATLAB Function  TreatAsAtomicUnit=on
  so_cha : Outport
  so_chb : Outport  Port=2
  wires:
  si_cha/1 -> sw_unit/1(si_cha)
  sw_unit/1(so_cha) -> out_dly_a/1
  out_dly_a/1 -> so_cha/1
  in_dly_b/1 -> sw_unit/2(si_chb)
  si_chb/1 -> in_dly_b/1
  sw_unit/2(so_chb) -> so_chb/1

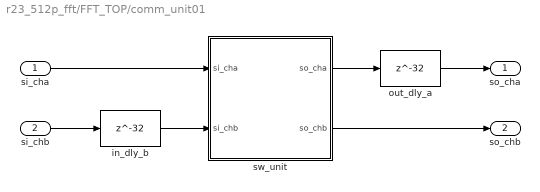
== system r23_512p_fft/FFT_TOP/comm_unit01 ==
  si_cha : Inport
  si_chb : Inport  Port=2
  in_dly_b : Delay  DelayLength=32
  out_dly_a : Delay  DelayLength=32
  sw_unit : MATLAB Function  TreatAsAtomicUnit=on
  so_cha : Outport
  so_chb : Outport  Port=2
  wires:
  sw_unit/2(so_chb) -> so_chb/1
  si_chb/1 -> in_dly_b/1
  in_dly_b/1 -> sw_unit/2(si_chb)
  out_dly_a/1 -> so_cha/1
  sw_unit/1(so_cha) -> out_dly_a/1
  si_cha/1 -> sw_unit/1(si_cha)

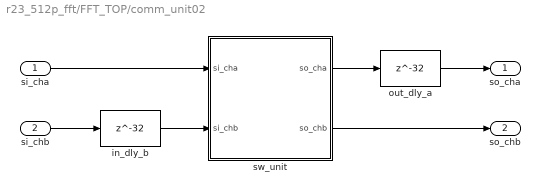
== system r23_512p_fft/FFT_TOP/comm_unit02 ==
  si_cha : Inport
  si_chb : Inport  Port=2
  in_dly_b : Delay  DelayLength=32
  out_dly_a : Delay  DelayLength=32
  sw_unit : MATLAB Function  TreatAsAtomicUnit=on
  so_cha : Outport
  so_chb : Outport  Port=2
  wires:
  si_cha/1 -> sw_unit/1(si_cha)
  sw_unit/1(so_cha) -> out_dly_a/1
  out_dly_a/1 -> so_cha/1
  in_dly_b/1 -> sw_unit/2(si_chb)
  si_chb/1 -> in_dly_b/1
  sw_unit/2(so_chb) -> so_chb/1

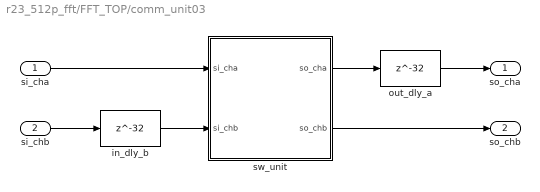
== system r23_512p_fft/FFT_TOP/comm_unit03 ==
  si_cha : Inport
  si_chb : Inport  Port=2
  in_dly_b : Delay  DelayLength=32
  out_dly_a : Delay  DelayLength=32
  sw_unit : MATLAB Function  TreatAsAtomicUnit=on
  so_cha : Outport
  so_chb : Outport  Port=2
  wires:
  sw_unit/2(so_chb) -> so_chb/1
  si_chb/1 -> in_dly_b/1
  in_dly_b/1 -> sw_unit/2(si_chb)
  out_dly_a/1 -> so_cha/1
  sw_unit/1(so_cha) -> out_dly_a/1
  si_cha/1 -> sw_unit/1(si_cha)

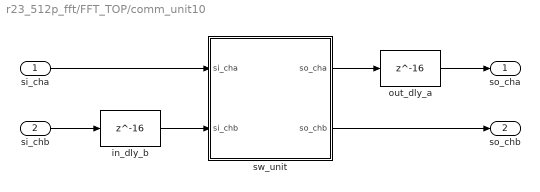
== system r23_512p_fft/FFT_TOP/comm_unit10 ==
  si_cha : Inport
  si_chb : Inport  Port=2
  in_dly_b : Delay  DelayLength=16
  out_dly_a : Delay  DelayLength=16
  sw_unit : MATLAB Function  TreatAsAtomicUnit=on
  so_cha : Outport
  so_chb : Outport  Port=2
  wires:
  sw_unit/2(so_chb) -> so_chb/1
  si_chb/1 -> in_dly_b/1
  in_dly_b/1 -> sw_unit/2(si_chb)
  out_dly_a/1 -> so_cha/1
  sw_unit/1(so_cha) -> out_dly_a/1
  si_cha/1 -> sw_unit/1(si_cha)

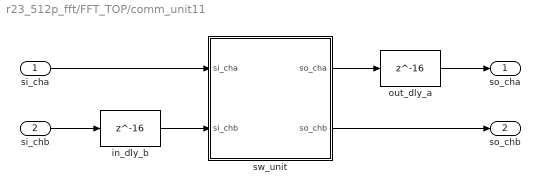
== system r23_512p_fft/FFT_TOP/comm_unit11 ==
  si_cha : Inport
  si_chb : Inport  Port=2
  in_dly_b : Delay  DelayLength=16
  out_dly_a : Delay  DelayLength=16
  sw_unit : MATLAB Function  TreatAsAtomicUnit=on
  so_cha : Outport
  so_chb : Outport  Port=2
  wires:
  si_cha/1 -> sw_unit/1(si_cha)
  sw_unit/1(so_cha) -> out_dly_a/1
  out_dly_a/1 -> so_cha/1
  in_dly_b/1 -> sw_unit/2(si_chb)
  si_chb/1 -> in_dly_b/1
  sw_unit/2(so_chb) -> so_chb/1

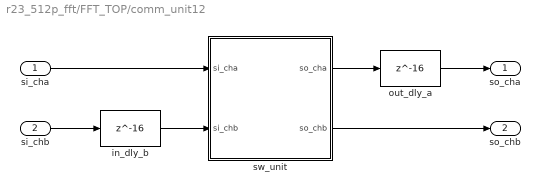
== system r23_512p_fft/FFT_TOP/comm_unit12 ==
  si_cha : Inport
  si_chb : Inport  Port=2
  in_dly_b : Delay  DelayLength=16
  out_dly_a : Delay  DelayLength=16
  sw_unit : MATLAB Function  TreatAsAtomicUnit=on
  so_cha : Outport
  so_chb : Outport  Port=2
  wires:
  sw_unit/2(so_chb) -> so_chb/1
  si_chb/1 -> in_dly_b/1
  in_dly_b/1 -> sw_unit/2(si_chb)
  out_dly_a/1 -> so_cha/1
  sw_unit/1(so_cha) -> out_dly_a/1
  si_cha/1 -> sw_unit/1(si_cha)

== system r23_512p_fft/FFT_TOP/comm_unit13 ==
  si_cha : Inport
  si_chb : Inport  Port=2
  in_dly_b : Delay  DelayLength=16
  out_dly_a : Delay  DelayLength=16
  sw_unit : MATLAB Function  TreatAsAtomicUnit=on
  so_cha : Outport
  so_chb : Outport  Port=2
  wires:
  si_cha/1 -> sw_unit/1(si_cha)
  sw_unit/1(so_cha) -> out_dly_a/1
  out_dly_a/1 -> so_cha/1
  in_dly_b/1 -> sw_unit/2(si_chb)
  si_chb/1 -> in_dly_b/1
  sw_unit/2(so_chb) -> so_chb/1

== system r23_512p_fft/FFT_TOP/comm_unit20 ==
  si_cha : Inport
  si_chb : Inport  Port=2
  in_dly_b : Delay  DelayLength=8
  out_dly_a : Delay  DelayLength=8
  sw_unit : MATLAB Function  TreatAsAtomicUnit=on
  so_cha : Outport
  so_chb : Outport  Port=2
  wires:
  si_cha/1 -> sw_unit/1(si_cha)
  sw_unit/1(so_cha) -> out_dly_a/1
  out_dly_a/1 -> so_cha/1
  in_dly_b/1 -> sw_unit/2(si_chb)
  si_chb/1 -> in_dly_b/1
  sw_unit/2(so_chb) -> so_chb/1

== system r23_512p_fft/FFT_TOP/comm_unit21 ==
  si_cha : Inport
  si_chb : Inport  Port=2
  in_dly_b : Delay  DelayLength=8
  out_dly_a : Delay  DelayLength=8
  sw_unit : MATLAB Function  TreatAsAtomicUnit=on
  so_cha : Outport
  so_chb : Outport  Port=2
  wires:
  sw_unit/2(so_chb) -> so_chb/1
  si_chb/1 -> in_dly_b/1
  in_dly_b/1 -> sw_unit/2(si_chb)
  out_dly_a/1 -> so_cha/1
  sw_unit/1(so_cha) -> out_dly_a/1
  si_cha/1 -> sw_unit/1(si_cha)

== system r23_512p_fft/FFT_TOP/comm_unit22 ==
  si_cha : Inport
  si_chb : Inport  Port=2
  in_dly_b : Delay  DelayLength=8
  out_dly_a : Delay  DelayLength=8
  sw_unit : MATLAB Function  TreatAsAtomicUnit=on
  so_cha : Outport
  so_chb : Outport  Port=2
  wires:
  si_cha/1 -> sw_unit/1(si_cha)
  sw_unit/1(so_cha) -> out_dly_a/1
  out_dly_a/1 -> so_cha/1
  in_dly_b/1 -> sw_unit/2(si_chb)
  si_chb/1 -> in_dly_b/1
  sw_unit/2(so_chb) -> so_chb/1

== system r23_512p_fft/FFT_TOP/comm_unit23 ==
  si_cha : Inport
  si_chb : Inport  Port=2
  in_dly_b : Delay  DelayLength=8
  out_dly_a : Delay  DelayLength=8
  sw_unit : MATLAB Function  TreatAsAtomicUnit=on
  so_cha : Outport
  so_chb : Outport  Port=2
  wires:
  sw_unit/2(so_chb) -> so_chb/1
  si_chb/1 -> in_dly_b/1
  in_dly_b/1 -> sw_unit/2(si_chb)
  out_dly_a/1 -> so_cha/1
  sw_unit/1(so_cha) -> out_dly_a/1
  si_cha/1 -> sw_unit/1(si_cha)

== system r23_512p_fft/FFT_TOP/comm_unit30 ==
  si_cha : Inport
  si_chb : Inport  Port=2
  in_dly_b : Delay  DelayLength=4
  out_dly_a : Delay  DelayLength=4
  sw_unit : MATLAB Function  TreatAsAtomicUnit=on
  so_cha : Outport
  so_chb : Outport  Port=2
  wires:
  sw_unit/2(so_chb) -> so_chb/1
  si_chb/1 -> in_dly_b/1
  in_dly_b/1 -> sw_unit/2(si_chb)
  out_dly_a/1 -> so_cha/1
  sw_unit/1(so_cha) -> out_dly_a/1
  si_cha/1 -> sw_unit/1(si_cha)

== system r23_512p_fft/FFT_TOP/comm_unit31 ==
  si_cha : Inport
  si_chb : Inport  Port=2
  in_dly_b : Delay  DelayLength=4
  out_dly_a : Delay  DelayLength=4
  sw_unit : MATLAB Function  TreatAsAtomicUnit=on
  so_cha : Outport
  so_chb : Outport  Port=2
  wires:
  si_cha/1 -> sw_unit/1(si_cha)
  sw_unit/1(so_cha) -> out_dly_a/1
  out_dly_a/1 -> so_cha/1
  in_dly_b/1 -> sw_unit/2(si_chb)
  si_chb/1 -> in_dly_b/1
  sw_unit/2(so_chb) -> so_chb/1

== system r23_512p_fft/FFT_TOP/comm_unit32 ==
  si_cha : Inport
  si_chb : Inport  Port=2
  in_dly_b : Delay  DelayLength=4
  out_dly_a : Delay  DelayLength=4
  sw_unit : MATLAB Function  TreatAsAtomicUnit=on
  so_cha : Outport
  so_chb : Outport  Port=2
  wires:
  sw_unit/2(so_chb) -> so_chb/1
  si_chb/1 -> in_dly_b/1
  in_dly_b/1 -> sw_unit/2(si_chb)
  out_dly_a/1 -> so_cha/1
  sw_unit/1(so_cha) -> out_dly_a/1
  si_cha/1 -> sw_unit/1(si_cha)

== system r23_512p_fft/FFT_TOP/comm_unit33 ==
  si_cha : Inport
  si_chb : Inport  Port=2
  in_dly_b : Delay  DelayLength=4
  out_dly_a : Delay  DelayLength=4
  sw_unit : MATLAB Function  TreatAsAtomicUnit=on
  so_cha : Outport
  so_chb : Outport  Port=2
  wires:
  si_cha/1 -> sw_unit/1(si_cha)
  sw_unit/1(so_cha) -> out_dly_a/1
  out_dly_a/1 -> so_cha/1
  in_dly_b/1 -> sw_unit/2(si_chb)
  si_chb/1 -> in_dly_b/1
  sw_unit/2(so_chb) -> so_chb/1

== system r23_512p_fft/FFT_TOP/comm_unit40 ==
  si_cha : Inport
  si_chb : Inport  Port=2
  in_dly_b : Delay
  out_dly_a : Delay
  sw_unit : MATLAB Function  TreatAsAtomicUnit=on
  so_cha : Outport
  so_chb : Outport  Port=2
  wires:
  si_cha/1 -> sw_unit/1(si_cha)
  sw_unit/1(so_cha) -> out_dly_a/1
  out_dly_a/1 -> so_cha/1
  in_dly_b/1 -> sw_unit/2(si_chb)
  si_chb/1 -> in_dly_b/1
  sw_unit/2(so_chb) -> so_chb/1

== system r23_512p_fft/FFT_TOP/comm_unit41 ==
  si_cha : Inport
  si_chb : Inport  Port=2
  in_dly_b : Delay
  out_dly_a : Delay
  sw_unit : MATLAB Function  TreatAsAtomicUnit=on
  so_cha : Outport
  so_chb : Outport  Port=2
  wires:
  sw_unit/2(so_chb) -> so_chb/1
  si_chb/1 -> in_dly_b/1
  in_dly_b/1 -> sw_unit/2(si_chb)
  out_dly_a/1 -> so_cha/1
  sw_unit/1(so_cha) -> out_dly_a/1
  si_cha/1 -> sw_unit/1(si_cha)

== system r23_512p_fft/FFT_TOP/comm_unit42 ==
  si_cha : Inport
  si_chb : Inport  Port=2
  in_dly_b : Delay
  out_dly_a : Delay
  sw_unit : MATLAB Function  TreatAsAtomicUnit=on
  so_cha : Outport
  so_chb : Outport  Port=2
  wires:
  si_cha/1 -> sw_unit/1(si_cha)
  sw_unit/1(so_cha) -> out_dly_a/1
  out_dly_a/1 -> so_cha/1
  in_dly_b/1 -> sw_unit/2(si_chb)
  si_chb/1 -> in_dly_b/1
  sw_unit/2(so_chb) -> so_chb/1

== system r23_512p_fft/FFT_TOP/comm_unit43 ==
  si_cha : Inport
  si_chb : Inport  Port=2
  in_dly_b : Delay
  out_dly_a : Delay
  sw_unit : MATLAB Function  TreatAsAtomicUnit=on
  so_cha : Outport
  so_chb : Outport  Port=2
  wires:
  sw_unit/2(so_chb) -> so_chb/1
  si_chb/1 -> in_dly_b/1
  in_dly_b/1 -> sw_unit/2(si_chb)
  out_dly_a/1 -> so_cha/1
  sw_unit/1(so_cha) -> out_dly_a/1
  si_cha/1 -> sw_unit/1(si_cha)

== system r23_512p_fft/FFT_TOP/comm_unit50 ==
  si_cha : Inport
  si_chb : Inport  Port=2
  in_dly_b : Delay  DelayLength=1
  out_dly_a : Delay  DelayLength=1
  sw_unit : MATLAB Function  TreatAsAtomicUnit=on
  so_cha : Outport
  so_chb : Outport  Port=2
  wires:
  sw_unit/2(so_chb) -> so_chb/1
  si_chb/1 -> in_dly_b/1
  in_dly_b/1 -> sw_unit/2(si_chb)
  out_dly_a/1 -> so_cha/1
  sw_unit/1(so_cha) -> out_dly_a/1
  si_cha/1 -> sw_unit/1(si_cha)

== system r23_512p_fft/FFT_TOP/comm_unit51 ==
  si_cha : Inport
  si_chb : Inport  Port=2
  in_dly_b : Delay  DelayLength=1
  out_dly_a : Delay  DelayLength=1
  sw_unit : MATLAB Function  TreatAsAtomicUnit=on
  so_cha : Outport
  so_chb : Outport  Port=2
  wires:
  si_cha/1 -> sw_unit/1(si_cha)
  sw_unit/1(so_cha) -> out_dly_a/1
  out_dly_a/1 -> so_cha/1
  in_dly_b/1 -> sw_unit/2(si_chb)
  si_chb/1 -> in_dly_b/1
  sw_unit/2(so_chb) -> so_chb/1

== system r23_512p_fft/FFT_TOP/comm_unit52 ==
  si_cha : Inport
  si_chb : Inport  Port=2
  in_dly_b : Delay  DelayLength=1
  out_dly_a : Delay  DelayLength=1
  sw_unit : MATLAB Function  TreatAsAtomicUnit=on
  so_cha : Outport
  so_chb : Outport  Port=2
  wires:
  sw_unit/2(so_chb) -> so_chb/1
  si_chb/1 -> in_dly_b/1
  in_dly_b/1 -> sw_unit/2(si_chb)
  out_dly_a/1 -> so_cha/1
  sw_unit/1(so_cha) -> out_dly_a/1
  si_cha/1 -> sw_unit/1(si_cha)

== system r23_512p_fft/FFT_TOP/comm_unit53 ==
  si_cha : Inport
  si_chb : Inport  Port=2
  in_dly_b : Delay  DelayLength=1
  out_dly_a : Delay  DelayLength=1
  sw_unit : MATLAB Function  TreatAsAtomicUnit=on
  so_cha : Outport
  so_chb : Outport  Port=2
  wires:
  si_cha/1 -> sw_unit/1(si_cha)
  sw_unit/1(so_cha) -> out_dly_a/1
  out_dly_a/1 -> so_cha/1
  in_dly_b/1 -> sw_unit/2(si_chb)
  si_chb/1 -> in_dly_b/1
  sw_unit/2(so_chb) -> so_chb/1

== matlab function r23_512p_fft/FFT_TOP/calc_unit16/r2_unit ==
  data: si_cha input; so_cha output; so_chb output; si_chb input
function [so_cha, so_chb] = r2_unit(si_cha, si_chb)
%R2_UNIT Radix-2 butterfly.

DW = 14;
fm = fimath('RoundingMethod', 'Nearest', 'OverflowAction', 'Saturate', ...
    'ProductMode', 'FullPrecision', 'SumMode', 'FullPrecision');

so_cha = fi(zeros(1, 2), 1, DW, 0, fm);
so_chb = fi(zeros(1, 2), 1, DW, 0, fm);
so_cha(:) = si_cha + si_chb;
so_chb(:) = si_cha - si_chb;
end

== matlab function r23_512p_fft/FFT_TOP/calc_unit12/r2_unit ==
  data: si_cha input; so_cha output; so_chb output; si_chb input
function [so_cha, so_chb] = r2_unit(si_cha, si_chb)
%R2_UNIT Radix-2 butterfly.

DW = 13;
fm = fimath('RoundingMethod', 'Nearest', 'OverflowAction', 'Saturate', ...
    'ProductMode', 'FullPrecision', 'SumMode', 'FullPrecision');

so_cha = fi(zeros(1, 2), 1, DW, 0, fm);
so_chb = fi(zeros(1, 2), 1, DW, 0, fm);
so_cha(:) = si_cha + si_chb;
so_chb(:) = si_cha - si_chb;
end

== matlab function r23_512p_fft/FFT_TOP/calc_unit11/r2_unit ==
  data: si_cha input; so_cha output; so_chb output; si_chb input
function [so_cha, so_chb] = r2_unit(si_cha, si_chb)
%R2_UNIT Radix-2 butterfly.

DW = 14;
fm = fimath('RoundingMethod', 'Nearest', 'OverflowAction', 'Saturate', ...
    'ProductMode', 'FullPrecision', 'SumMode', 'FullPrecision');

so_cha = fi(zeros(1, 2), 1, DW, 0, fm);
so_chb = fi(zeros(1, 2), 1, DW, 0, fm);
so_cha(:) = si_cha + si_chb;
so_chb(:) = si_cha - si_chb;
end

== matlab function r23_512p_fft/FFT_TOP/calc_unit19/r2_unit ==
  data: si_cha input; so_cha output; so_chb output; si_chb input
function [so_cha, so_chb] = r2_unit(si_cha, si_chb)
%R2_UNIT Radix-2 butterfly.

DW = 14;
fm = fimath('RoundingMethod', 'Nearest', 'OverflowAction', 'Saturate', ...
    'ProductMode', 'FullPrecision', 'SumMode', 'FullPrecision');

so_cha = fi(zeros(1, 2), 1, DW, 0, fm);
so_chb = fi(zeros(1, 2), 1, DW, 0, fm);
so_cha(:) = si_cha + si_chb;
so_chb(:) = si_cha - si_chb;
end

== matlab function r23_512p_fft/FFT_TOP/calc_unit18/r2_unit ==
  data: si_cha input; so_cha output; so_chb output; si_chb input
function [so_cha, so_chb] = r2_unit(si_cha, si_chb)
%R2_UNIT Radix-2 butterfly.

DW = 14;
fm = fimath('RoundingMethod', 'Nearest', 'OverflowAction', 'Saturate', ...
    'ProductMode', 'FullPrecision', 'SumMode', 'FullPrecision');

so_cha = fi(zeros(1, 2), 1, DW, 0, fm);
so_chb = fi(zeros(1, 2), 1, DW, 0, fm);
so_cha(:) = si_cha + si_chb;
so_chb(:) = si_cha - si_chb;
end

== matlab function r23_512p_fft/FFT_TOP/calc_unit17/r2_unit ==
  data: si_cha input; so_cha output; so_chb output; si_chb input
function [so_cha, so_chb] = r2_unit(si_cha, si_chb)
%R2_UNIT Radix-2 butterfly.

DW = 14;
fm = fimath('RoundingMethod', 'Nearest', 'OverflowAction', 'Saturate', ...
    'ProductMode', 'FullPrecision', 'SumMode', 'FullPrecision');

so_cha = fi(zeros(1, 2), 1, DW, 0, fm);
so_chb = fi(zeros(1, 2), 1, DW, 0, fm);
so_cha(:) = si_cha + si_chb;
so_chb(:) = si_cha - si_chb;
end

== matlab function r23_512p_fft/FFT_TOP/calc_unit22/r2_unit ==
  data: si_cha input; so_cha output; so_chb output; si_chb input
function [so_cha, so_chb] = r2_unit(si_cha, si_chb)
%R2_UNIT Radix-2 butterfly.

DW = 15;
fm = fimath('RoundingMethod', 'Nearest', 'OverflowAction', 'Saturate', ...
    'ProductMode', 'FullPrecision', 'SumMode', 'FullPrecision');

so_cha = fi(zeros(1, 2), 1, DW, 0, fm);
so_chb = fi(zeros(1, 2), 1, DW, 0, fm);
so_cha(:) = si_cha + si_chb;
so_chb(:) = si_cha - si_chb;
end

== matlab function r23_512p_fft/FFT_TOP/calc_unit23/r2_unit ==
  data: si_cha input; so_cha output; so_chb output; si_chb input
function [so_cha, so_chb] = r2_unit(si_cha, si_chb)
%R2_UNIT Radix-2 butterfly.

DW = 15;
fm = fimath('RoundingMethod', 'Nearest', 'OverflowAction', 'Saturate', ...
    'ProductMode', 'FullPrecision', 'SumMode', 'FullPrecision');

so_cha = fi(zeros(1, 2), 1, DW, 0, fm);
so_chb = fi(zeros(1, 2), 1, DW, 0, fm);
so_cha(:) = si_cha + si_chb;
so_chb(:) = si_cha - si_chb;
end

== matlab function r23_512p_fft/FFT_TOP/calc_unit20/r2_unit ==
  data: si_cha input; so_cha output; so_chb output; si_chb input
function [so_cha, so_chb] = r2_unit(si_cha, si_chb)
%R2_UNIT Radix-2 butterfly.

DW = 15;
fm = fimath('RoundingMethod', 'Nearest', 'OverflowAction', 'Saturate', ...
    'ProductMode', 'FullPrecision', 'SumMode', 'FullPrecision');

so_cha = fi(zeros(1, 2), 1, DW, 0, fm);
so_chb = fi(zeros(1, 2), 1, DW, 0, fm);
so_cha(:) = si_cha + si_chb;
so_chb(:) = si_cha - si_chb;
end

== matlab function r23_512p_fft/FFT_TOP/calc_unit21/r2_unit ==
  data: si_cha input; so_cha output; so_chb output; si_chb input
function [so_cha, so_chb] = r2_unit(si_cha, si_chb)
%R2_UNIT Radix-2 butterfly.

DW = 15;
fm = fimath('RoundingMethod', 'Nearest', 'OverflowAction', 'Saturate', ...
    'ProductMode', 'FullPrecision', 'SumMode', 'FullPrecision');

so_cha = fi(zeros(1, 2), 1, DW, 0, fm);
so_chb = fi(zeros(1, 2), 1, DW, 0, fm);
so_cha(:) = si_cha + si_chb;
so_chb(:) = si_cha - si_chb;
end

== matlab function r23_512p_fft/FFT_TOP/calc_unit24/r2_unit ==
  data: si_cha input; so_cha output; so_chb output; si_chb input
function [so_cha, so_chb] = r2_unit(si_cha, si_chb)
%R2_UNIT Radix-2 butterfly.

DW = 14;
fm = fimath('RoundingMethod', 'Nearest', 'OverflowAction', 'Saturate', ...
    'ProductMode', 'FullPrecision', 'SumMode', 'FullPrecision');

so_cha = fi(zeros(1, 2), 1, DW, 0, fm);
so_chb = fi(zeros(1, 2), 1, DW, 0, fm);
so_cha(:) = si_cha + si_chb;
so_chb(:) = si_cha - si_chb;
end

== matlab function r23_512p_fft/FFT_TOP/calc_unit25/r2_unit ==
  data: si_cha input; so_cha output; so_chb output; si_chb input
function [so_cha, so_chb] = r2_unit(si_cha, si_chb)
%R2_UNIT Radix-2 butterfly.

DW = 14;
fm = fimath('RoundingMethod', 'Nearest', 'OverflowAction', 'Saturate', ...
    'ProductMode', 'FullPrecision', 'SumMode', 'FullPrecision');

so_cha = fi(zeros(1, 2), 1, DW, 0, fm);
so_chb = fi(zeros(1, 2), 1, DW, 0, fm);
so_cha(:) = si_cha + si_chb;
so_chb(:) = si_cha - si_chb;
end

== matlab function r23_512p_fft/FFT_TOP/calc_unit13/r2_unit ==
  data: si_cha input; so_cha output; so_chb output; si_chb input
function [so_cha, so_chb] = r2_unit(si_cha, si_chb)
%R2_UNIT Radix-2 butterfly.

DW = 13;
fm = fimath('RoundingMethod', 'Nearest', 'OverflowAction', 'Saturate', ...
    'ProductMode', 'FullPrecision', 'SumMode', 'FullPrecision');

so_cha = fi(zeros(1, 2), 1, DW, 0, fm);
so_chb = fi(zeros(1, 2), 1, DW, 0, fm);
so_cha(:) = si_cha + si_chb;
so_chb(:) = si_cha - si_chb;
end

== matlab function r23_512p_fft/FFT_TOP/calc_unit26/r2_unit ==
  data: si_cha input; so_cha output; so_chb output; si_chb input
function [so_cha, so_chb] = r2_unit(si_cha, si_chb)
%R2_UNIT Radix-2 butterfly.

DW = 14;
fm = fimath('RoundingMethod', 'Nearest', 'OverflowAction', 'Saturate', ...
    'ProductMode', 'FullPrecision', 'SumMode', 'FullPrecision');

so_cha = fi(zeros(1, 2), 1, DW, 0, fm);
so_chb = fi(zeros(1, 2), 1, DW, 0, fm);
so_cha(:) = si_cha + si_chb;
so_chb(:) = si_cha - si_chb;
end

== matlab function r23_512p_fft/FFT_TOP/calc_unit27/r2_unit ==
  data: si_cha input; so_cha output; so_chb output; si_chb input
function [so_cha, so_chb] = r2_unit(si_cha, si_chb)
%R2_UNIT Radix-2 butterfly.

DW = 14;
fm = fimath('RoundingMethod', 'Nearest', 'OverflowAction', 'Saturate', ...
    'ProductMode', 'FullPrecision', 'SumMode', 'FullPrecision');

so_cha = fi(zeros(1, 2), 1, DW, 0, fm);
so_chb = fi(zeros(1, 2), 1, DW, 0, fm);
so_cha(:) = si_cha + si_chb;
so_chb(:) = si_cha - si_chb;
end

== matlab function r23_512p_fft/FFT_TOP/calc_unit28/r2_unit ==
  data: si_cha input; so_cha output; so_chb output; si_chb input
function [so_cha, so_chb] = r2_unit(si_cha, si_chb)
%R2_UNIT Radix-2 butterfly.

DW = 15;
fm = fimath('RoundingMethod', 'Nearest', 'OverflowAction', 'Saturate', ...
    'ProductMode', 'FullPrecision', 'SumMode', 'FullPrecision');

so_cha = fi(zeros(1, 2), 1, DW, 0, fm);
so_chb = fi(zeros(1, 2), 1, DW, 0, fm);
so_cha(:) = si_cha + si_chb;
so_chb(:) = si_cha - si_chb;
end

== matlab function r23_512p_fft/FFT_TOP/calc_unit31/r2_unit ==
  data: si_cha input; so_cha output; so_chb output; si_chb input
function [so_cha, so_chb] = r2_unit(si_cha, si_chb)
%R2_UNIT Radix-2 butterfly.

DW = 15;
fm = fimath('RoundingMethod', 'Nearest', 'OverflowAction', 'Saturate', ...
    'ProductMode', 'FullPrecision', 'SumMode', 'FullPrecision');

so_cha = fi(zeros(1, 2), 1, DW, 0, fm);
so_chb = fi(zeros(1, 2), 1, DW, 0, fm);
so_cha(:) = si_cha + si_chb;
so_chb(:) = si_cha - si_chb;
end

== matlab function r23_512p_fft/FFT_TOP/calc_unit30/r2_unit ==
  data: si_cha input; so_cha output; so_chb output; si_chb input
function [so_cha, so_chb] = r2_unit(si_cha, si_chb)
%R2_UNIT Radix-2 butterfly.

DW = 15;
fm = fimath('RoundingMethod', 'Nearest', 'OverflowAction', 'Saturate', ...
    'ProductMode', 'FullPrecision', 'SumMode', 'FullPrecision');

so_cha = fi(zeros(1, 2), 1, DW, 0, fm);
so_chb = fi(zeros(1, 2), 1, DW, 0, fm);
so_cha(:) = si_cha + si_chb;
so_chb(:) = si_cha - si_chb;
end
